simulink model "ecmOffline"  (R2025b)
settings: Solver=ode45  StartTime=0.0  StopTime=600  MaxStep=ECM.Ts  RelTol=1e-6  AbsTol=1e-8
InitFcn:
  | if ~exist('ECM','var'), ECM = ecmParams; end
values from neighbouring files (symbols this model uses):
  ECM = ecmParams(TempDep=false, Degradation=false, IC=struct("soc0", zD(1, :), "T0C", mean(tC(1, :))))    [checkFastPlant.m]
settings Model: SimulationMode=accelerator  Creator=SC-Br  LastModifiedBy=SC-Br
settings DataIOCC: SaveFinalState=on  SaveOperatingPoint=on  SaveOutput=off  SignalLogging=off  SaveTime=off
settings DebuggingCC: AlgebraicLoopMsg=error  UnconnectedInputMsg=error

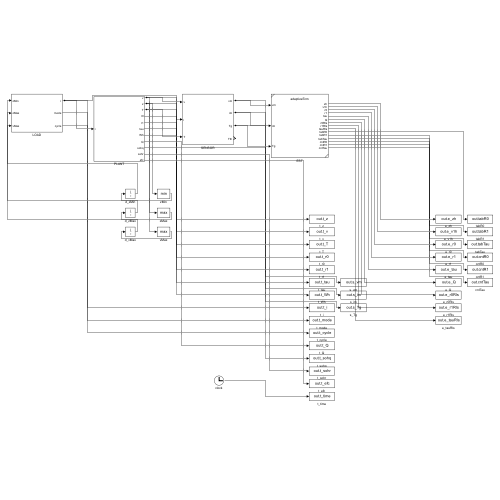
[thumbnail: Simulink's stored preview of the top-level diagram]
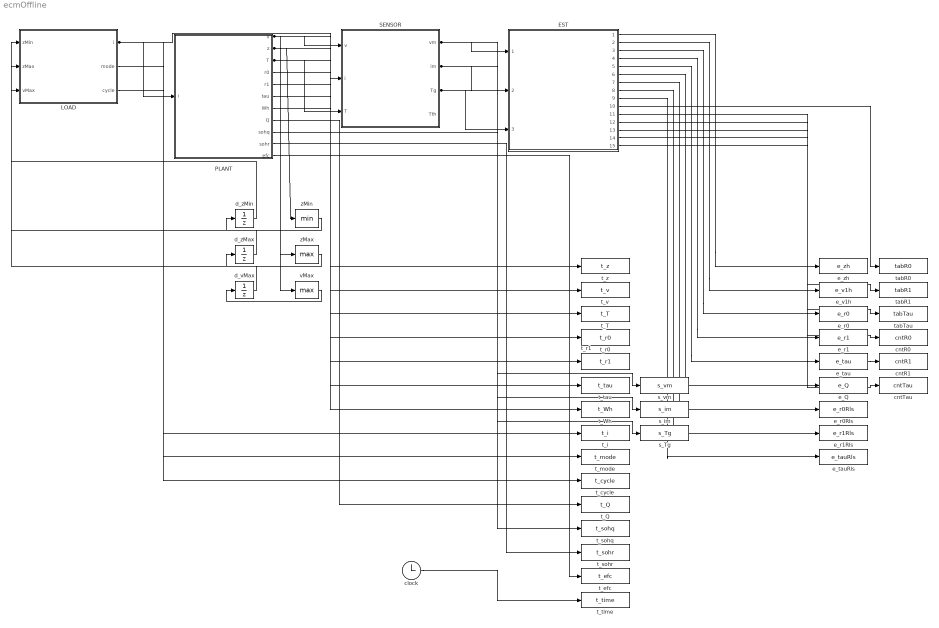
== system ecmOffline ==
  EST : Subsystem  ReferencedSubsystem=adaptiveEcm
  LOAD : Subsystem
  PLANT : Subsystem
  SENSOR : Subsystem
  clock : Clock
  cntR0 : ToWorkspace  VariableName=cntR0  SaveFormat=Structure With Time  SampleTime=ECM.TsLog
      settings: MaxDataPoints=1
  cntR1 : ToWorkspace  VariableName=cntR1  SaveFormat=Structure With Time  SampleTime=ECM.TsLog
      settings: MaxDataPoints=1
  cntTau : ToWorkspace  VariableName=cntTau  SaveFormat=Structure With Time  SampleTime=ECM.TsLog
      settings: MaxDataPoints=1
  d_vMax : UnitDelay  SampleTime=ECM.Ts  HasFrameUpgradeWarning=on
  d_zMax : UnitDelay  InitialCondition=max(ECM.plant.soc0)  SampleTime=ECM.Ts  HasFrameUpgradeWarning=on
  d_zMin : UnitDelay  InitialCondition=min(ECM.plant.soc0)  SampleTime=ECM.Ts  HasFrameUpgradeWarning=on
  e_Q : ToWorkspace  VariableName=e_Q  SampleTime=ECM.TsLog
  e_r0 : ToWorkspace  VariableName=e_r0  SampleTime=ECM.TsLog
  e_r0Rls : ToWorkspace  VariableName=e_r0Rls  SampleTime=ECM.TsLog
  e_r1 : ToWorkspace  VariableName=e_r1  SampleTime=ECM.TsLog
  e_r1Rls : ToWorkspace  VariableName=e_r1Rls  SampleTime=ECM.TsLog
  e_tau : ToWorkspace  VariableName=e_tau  SampleTime=ECM.TsLog
  e_tauRls : ToWorkspace  VariableName=e_tauRls  SampleTime=ECM.TsLog
  e_v1h : ToWorkspace  VariableName=e_v1h  SampleTime=ECM.TsLog
  e_zh : ToWorkspace  VariableName=e_zh  SampleTime=ECM.TsLog
  s_Tg : ToWorkspace  VariableName=s_Tg  SampleTime=ECM.Ts
      settings: MaxDataPoints=ECM.logSensorPoints
  s_im : ToWorkspace  VariableName=s_im  SampleTime=ECM.Ts
      settings: MaxDataPoints=ECM.logSensorPoints
  s_vm : ToWorkspace  VariableName=s_vm  SampleTime=ECM.Ts
      settings: MaxDataPoints=ECM.logSensorPoints
  t_Q : ToWorkspace  VariableName=t_Q  SampleTime=ECM.TsLog
  t_T : ToWorkspace  VariableName=t_T  SampleTime=ECM.TsLog
  t_Wh : ToWorkspace  VariableName=t_Wh  SampleTime=ECM.TsLog
  t_cycle : ToWorkspace  VariableName=t_cycle  SampleTime=ECM.TsLog
  t_efc : ToWorkspace  VariableName=t_efc  SampleTime=ECM.TsLog
  t_i : ToWorkspace  VariableName=t_i  SampleTime=ECM.TsLog
  t_mode : ToWorkspace  VariableName=t_mode  SampleTime=ECM.TsLog
  t_r0 : ToWorkspace  VariableName=t_r0  SampleTime=ECM.TsLog
  t_r1 : ToWorkspace  VariableName=t_r1  SampleTime=ECM.TsLog
  t_sohq : ToWorkspace  VariableName=t_sohq  SampleTime=ECM.TsLog
  t_sohr : ToWorkspace  VariableName=t_sohr  SampleTime=ECM.TsLog
  t_tau : ToWorkspace  VariableName=t_tau  SampleTime=ECM.TsLog
  t_time : ToWorkspace  VariableName=t_time  SampleTime=ECM.TsLog
  t_v : ToWorkspace  VariableName=t_v  SampleTime=ECM.TsLog
  t_z : ToWorkspace  VariableName=t_z  SampleTime=ECM.TsLog
  tabR0 : ToWorkspace  VariableName=tabR0  SaveFormat=Structure With Time  SampleTime=ECM.TsLog
      settings: MaxDataPoints=1
  tabR1 : ToWorkspace  VariableName=tabR1  SaveFormat=Structure With Time  SampleTime=ECM.TsLog
      settings: MaxDataPoints=1
  tabTau : ToWorkspace  VariableName=tabTau  SaveFormat=Structure With Time  SampleTime=ECM.TsLog
      settings: MaxDataPoints=1
  vMax : MinMax  Function=max
  zMax : MinMax  Function=max
  zMin : MinMax
  wires:
  LOAD/1(i) -> PLANT/1(i), SENSOR/2(i), t_i/1
  PLANT/1(v) -> SENSOR/1(v), vMax/1, t_v/1
  PLANT/3(T) -> SENSOR/3(T), t_T/1
  PLANT/2(z) -> zMin/1, zMax/1, t_z/1
  zMin/1 -> d_zMin/1
  d_zMin/1 -> LOAD/1(zMin)
  zMax/1 -> d_zMax/1
  d_zMax/1 -> LOAD/2(zMax)
  vMax/1 -> d_vMax/1
  d_vMax/1 -> LOAD/3(vMax)
  SENSOR/1(vm) -> EST/1, s_vm/1
  SENSOR/2(im) -> EST/2, s_im/1
  SENSOR/3(Tg) -> EST/3, s_Tg/1
  PLANT/4(r0) -> t_r0/1
  PLANT/5(r1) -> t_r1/1
  PLANT/6(tau) -> t_tau/1
  PLANT/7(Wh) -> t_Wh/1
  LOAD/2(mode) -> t_mode/1
  LOAD/3(cycle) -> t_cycle/1
  PLANT/8(Q) -> t_Q/1
  PLANT/9(sohq) -> t_sohq/1
  PLANT/10(sohr) -> t_sohr/1
  PLANT/11(efc) -> t_efc/1
  clock/1 -> t_time/1
  EST/1 -> e_zh/1
  EST/2 -> e_v1h/1
  EST/3 -> e_r0/1
  EST/4 -> e_r1/1
  EST/5 -> e_tau/1
  EST/6 -> e_Q/1
  EST/7 -> e_r0Rls/1
  EST/8 -> e_r1Rls/1
  EST/9 -> e_tauRls/1
  EST/10 -> tabR0/1
  EST/11 -> tabR1/1
  EST/12 -> tabTau/1
  EST/13 -> cntR0/1
  EST/14 -> cntR1/1
  EST/15 -> cntTau/1

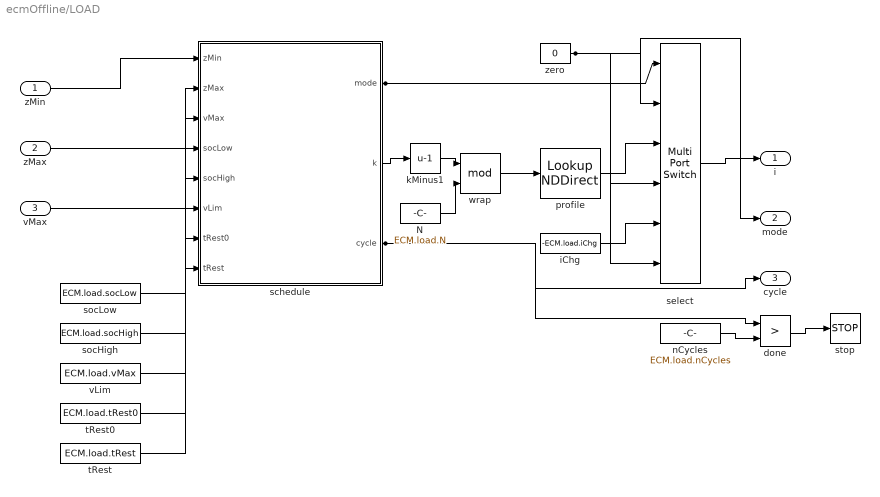
== system ecmOffline/LOAD ==
  zMin : Inport
  zMax : Inport  Port=2
  vMax : Inport  Port=3
  N : Constant  Value=ECM.load.N
  done : RelationalOperator  Operator=>  OutDataTypeStr=boolean  RndMeth=Simplest  InputSameDT=off
  iChg : Constant  Value=-ECM.load.iChg
  kMinus1 : Bias  Bias=-1  SaturateOnIntegerOverflow=off
  nCycles : Constant  Value=ECM.load.nCycles
  profile : LookupNDDirect  NumberOfTableDimensions=1  Table=ECM.load.profile
  schedule : Stateflow chart  TreatAsAtomicUnit=on
  select : MultiPortSwitch  DataPortOrder=Zero-based contiguous  Inputs=5  zeroidx=on  SaturateOnIntegerOverflow=off  InputSameDT=off
  socHigh : Constant  Value=ECM.load.socHigh
  socLow : Constant  Value=ECM.load.socLow
  stop : Stop
  tRest : Constant  Value=ECM.load.tRest
  tRest0 : Constant  Value=ECM.load.tRest0
  vLim : Constant  Value=ECM.load.vMax
  wrap : Math  Operator=mod
  zero : Constant  Value=0
  i : Outport
  mode : Outport  Port=2
  cycle : Outport  Port=3
  wires:
  zMin/1 -> schedule/1(zMin)
  zMax/1 -> schedule/2(zMax)
  vMax/1 -> schedule/3(vMax)
  socLow/1 -> schedule/4(socLow)
  socHigh/1 -> schedule/5(socHigh)
  vLim/1 -> schedule/6(vLim)
  tRest0/1 -> schedule/7(tRest0)
  tRest/1 -> schedule/8(tRest)
  schedule/2(k) -> kMinus1/1
  kMinus1/1 -> wrap/1
  N/1 -> wrap/2
  wrap/1 -> profile/1
  schedule/1(mode) -> select/1, mode/1
  zero/1 -> select/2, select/4, select/6
  profile/1 -> select/3
  iChg/1 -> select/5
  schedule/3(cycle) -> cycle/1, done/1
  nCycles/1 -> done/2
  done/1 -> stop/1
  select/1 -> i/1

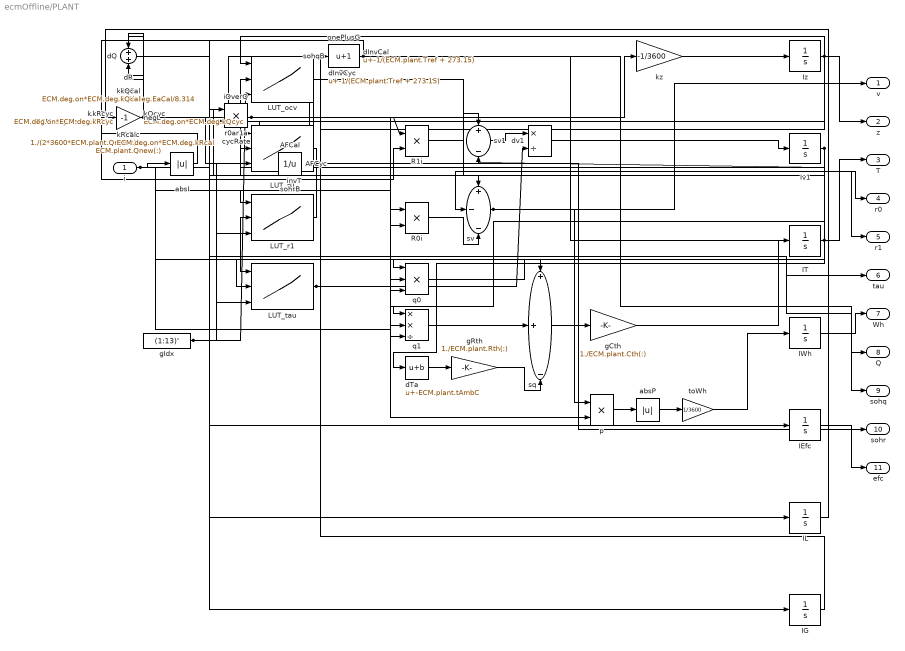
== system ecmOffline/PLANT ==
  i : Inport
  AFCal : Math
  AFCyc : Math
  IEfc : Integrator  InitialCondition=ECM.plant.efc0(:)
  IG : Integrator  InitialCondition=ECM.plant.G0(:)
  IL : Integrator  InitialCondition=ECM.plant.L0(:)
  IT : Integrator  InitialCondition=ECM.plant.T0C(:)
  IWh : Integrator  InitialCondition=zeros(13,1)
  Iv1 : Integrator  InitialCondition=zeros(13,1)
  Iz : Integrator  InitialCondition=ECM.plant.soc0(:)
  LUT_ocv : Lookup_n-D  NumberOfTableDimensions=3  BreakpointsForDimension1=ECM.plant.socBp  BreakpointsForDimension2=ECM.plant.tBpC  BreakpointsForDimension3=1:13  Table=ECM.plant.ocv  ExtrapMethod=Clip  UseLastTableValue=on  InternalRulePriority=Speed  RndMeth=Simplest
      settings: InputPortMap=u0,u1,u2
  LUT_r0 : Lookup_n-D  NumberOfTableDimensions=3  BreakpointsForDimension1=ECM.plant.socBp  BreakpointsForDimension2=ECM.plant.tBpC  BreakpointsForDimension3=1:13  Table=ECM.plant.r0  ExtrapMethod=Clip  UseLastTableValue=on  InternalRulePriority=Speed  RndMeth=Simplest
      settings: InputPortMap=u0,u1,u2
  LUT_r1 : Lookup_n-D  NumberOfTableDimensions=3  BreakpointsForDimension1=ECM.plant.socBp  BreakpointsForDimension2=ECM.plant.tBpC  BreakpointsForDimension3=1:13  Table=ECM.plant.r1  ExtrapMethod=Clip  UseLastTableValue=on  InternalRulePriority=Speed  RndMeth=Simplest
      settings: InputPortMap=u0,u1,u2
  LUT_tau : Lookup_n-D  NumberOfTableDimensions=3  BreakpointsForDimension1=ECM.plant.socBp  BreakpointsForDimension2=ECM.plant.tBpC  BreakpointsForDimension3=1:13  Table=ECM.plant.tau  ExtrapMethod=Clip  UseLastTableValue=on  InternalRulePriority=Speed  RndMeth=Simplest
      settings: InputPortMap=u0,u1,u2
  QnowB : Gain  Gain=ECM.plant.Qnew(:)
  R0i : Product
  R1i : Product
  TK : Bias  Bias=273.15  SaturateOnIntegerOverflow=off
  absI : Abs  SaturateOnIntegerOverflow=off
  absP : Abs  SaturateOnIntegerOverflow=off
  cycRate : Product
  dInvCal : Bias  Bias=-1/(ECM.plant.Tref + 273.15)  SaturateOnIntegerOverflow=off
  dInvCyc : Bias  Bias=-1/(ECM.plant.Tref + 273.15)  SaturateOnIntegerOverflow=off
  dQ : Sum
  dR : Sum
  dTa : Bias  Bias=-ECM.plant.tAmbC  SaturateOnIntegerOverflow=off
  dv1 : Product  Inputs=*/
  gCth : Gain  Gain=1./ECM.plant.Cth(:)
  gIdx : Constant  Value=(1:13)'
  gRth : Gain  Gain=1./ECM.plant.Rth(:)
  iOverQ : Product  Inputs=*/
  invT : Math  Operator=reciprocal
  kAFCal : Gain  Gain=-ECM.deg.EaCal/8.314
  kAFCyc : Gain  Gain=-ECM.deg.EaCyc/8.314
  kEfc : Gain  Gain=1./(2*3600*ECM.plant.Qnew(:))
  kQcal : Gain  Gain=ECM.deg.on*ECM.deg.kQcal
  kQcyc : Gain  Gain=ECM.deg.on*ECM.deg.kQcyc
  kRcal : Gain  Gain=ECM.deg.on*ECM.deg.kRcal
  kRcyc : Gain  Gain=ECM.deg.on*ECM.deg.kRcyc
  kz : Gain  Gain=-1/3600
  negL : Gain  Gain=-1
  onePlusG : Bias  Bias=1  SaturateOnIntegerOverflow=off
  p : Product
  q0 : Product  Inputs=***
  q1 : Product  Inputs=**/
  r0a : Product
  r1a : Product
  sohqB : Bias  Bias=1  SaturateOnIntegerOverflow=off
  sohrB : Math  Operator=reciprocal
  sq : Sum  Inputs=++-
  sv : Sum  Inputs=+--
  sv1 : Sum  Inputs=+-
  toWh : Gain  Gain=1/3600
  v : Outport
  z : Outport  Port=2
  T : Outport  Port=3
  r0 : Outport  Port=4
  r1 : Outport  Port=5
  tau : Outport  Port=6
  Wh : Outport  Port=7
  Q : Outport  Port=8
  sohq : Outport  Port=9
  sohr : Outport  Port=10
  efc : Outport  Port=11
  wires:
  Iz/1 -> LUT_ocv/1, LUT_r0/1, LUT_r1/1, LUT_tau/1, z/1
  IT/1 -> LUT_ocv/2, LUT_r0/2, LUT_r1/2, LUT_tau/2, TK/1, dTa/1, T/1
  gIdx/1 -> LUT_ocv/3, LUT_r0/3, LUT_r1/3, LUT_tau/3
  IG/1 -> onePlusG/1
  LUT_r0/1 -> r0a/1
  onePlusG/1 -> r0a/2, r1a/2, sohrB/1
  LUT_r1/1 -> r1a/1
  IL/1 -> negL/1
  negL/1 -> sohqB/1
  sohqB/1 -> QnowB/1, sohq/1
  i/1 -> iOverQ/1, absI/1, R1i/2, R0i/2, q0/1, q0/2, p/2
  QnowB/1 -> iOverQ/2, Q/1
  iOverQ/1 -> kz/1
  kz/1 -> Iz/1
  absI/1 -> kEfc/1
  kEfc/1 -> IEfc/1, cycRate/1
  TK/1 -> invT/1
  invT/1 -> dInvCyc/1, dInvCal/1
  dInvCyc/1 -> kAFCyc/1
  kAFCyc/1 -> AFCyc/1
  dInvCal/1 -> kAFCal/1
  kAFCal/1 -> AFCal/1
  AFCyc/1 -> cycRate/2
  cycRate/1 -> kQcyc/1, kRcyc/1
  AFCal/1 -> kQcal/1, kRcal/1
  kQcyc/1 -> dQ/1
  kQcal/1 -> dQ/2
  kRcyc/1 -> dR/1
  kRcal/1 -> dR/2
  dQ/1 -> IL/1
  dR/1 -> IG/1
  r1a/1 -> R1i/1, q1/3, r1/1
  R1i/1 -> sv1/1
  Iv1/1 -> sv1/2, sv/2, q1/1, q1/2
  sv1/1 -> dv1/1
  LUT_tau/1 -> dv1/2, tau/1
  dv1/1 -> Iv1/1
  r0a/1 -> R0i/1, q0/3, r0/1
  LUT_ocv/1 -> sv/1
  R0i/1 -> sv/3
  dTa/1 -> gRth/1
  q0/1 -> sq/1
  q1/1 -> sq/2
  gRth/1 -> sq/3
  sq/1 -> gCth/1
  gCth/1 -> IT/1
  sv/1 -> p/1, v/1
  p/1 -> absP/1
  absP/1 -> toWh/1
  toWh/1 -> IWh/1
  IWh/1 -> Wh/1
  sohrB/1 -> sohr/1
  IEfc/1 -> efc/1

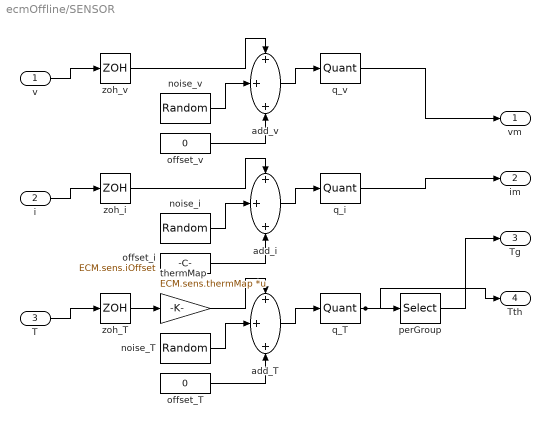
== system ecmOffline/SENSOR ==
  v : Inport
  i : Inport  Port=2
  T : Inport  Port=3
  add_T : Sum  Inputs=+++
  add_i : Sum  Inputs=+++
  add_v : Sum  Inputs=+++
  noise_T : RandomNumber  Mean=zeros(7,1)  Variance=ECM.sens.tNoise^2  Seed=ECM.sens.noiseSeed+3  SampleTime=ECM.Ts
  noise_i : RandomNumber  Mean=zeros(1,1)  Variance=ECM.sens.iNoise^2  Seed=ECM.sens.noiseSeed+2  SampleTime=ECM.Ts
  noise_v : RandomNumber  Mean=zeros(13,1)  Variance=ECM.sens.vNoise^2  Seed=ECM.sens.noiseSeed+1  SampleTime=ECM.Ts
  offset_T : Constant  Value=0
  offset_i : Constant  Value=ECM.sens.iOffset
  offset_v : Constant  Value=0
  perGroup : Selector  InputPortWidth=7  IndexOptions=Index vector (dialog)  Indices=ECM.sens.groupTherm  OutputSizes=1
  q_T : Quantizer  QuantizationInterval=ECM.sens.tLsb
  q_i : Quantizer  QuantizationInterval=ECM.sens.iLsb
  q_v : Quantizer  QuantizationInterval=ECM.sens.vLsb
  thermMap : Gain  Gain=ECM.sens.thermMap  Multiplication=Matrix(K*u)
  zoh_T : ZeroOrderHold  SampleTime=ECM.Ts
  zoh_i : ZeroOrderHold  SampleTime=ECM.Ts
  zoh_v : ZeroOrderHold  SampleTime=ECM.Ts
  vm : Outport
  im : Outport  Port=2
  Tg : Outport  Port=3
  Tth : Outport  Port=4
  wires:
  v/1 -> zoh_v/1
  zoh_v/1 -> add_v/1
  noise_v/1 -> add_v/2
  offset_v/1 -> add_v/3
  add_v/1 -> q_v/1
  i/1 -> zoh_i/1
  zoh_i/1 -> add_i/1
  noise_i/1 -> add_i/2
  offset_i/1 -> add_i/3
  add_i/1 -> q_i/1
  T/1 -> zoh_T/1
  zoh_T/1 -> thermMap/1
  thermMap/1 -> add_T/1
  noise_T/1 -> add_T/2
  offset_T/1 -> add_T/3
  add_T/1 -> q_T/1
  q_T/1 -> perGroup/1, Tth/1
  q_v/1 -> vm/1
  q_i/1 -> im/1
  perGroup/1 -> Tg/1

== stateflow chart ecmOffline/LOAD/schedule ==
  settings: updateMethod=DISCRETE  sampleTime=ECM.Ts
  state REST0
    entry: mode = 0;
  state DIS
    entry: mode = 1; k = k + 1;
    during: k = k + 1;
  state REST
    entry: mode = 2;
  state REST2
    entry: mode = 4;
  state CHG
    entry: mode = 3;
  (default) -> REST0
  DIS -> REST : [zMin <= socLow]
  REST0 -> DIS : after(tRest0,sec){cycle = 1;}
  REST2 -> DIS : after(tRest,sec){cycle = cycle + 1;}
  REST -> CHG : after(tRest,sec)
  CHG -> REST2 : [zMax >= socHigh || vMax >= vLim]
  data: zMin input; zMax input; vMax input; socLow input; socHigh input; vLim input; tRest0 input; tRest input; mode output =0; k output =0; cycle output =0
